simulink model "Ex-14050714-02_Hamming_Simulimk"  (R2025b)
settings: Solver=VariableStepDiscrete  StartTime=0.0  StopTime=1000  RelTol=1e-3
libraries: commblkcod2 x2, commrandsrc3 x1, commchan3 x1, commsink2 x1
settings Model: Creator=Pinnacle  LastModifiedBy=Pinnacle
settings SolverCC: AlgebraicLoopSolver=TrustRegion
settings DataIOCC: LimitDataPoints=on  SaveOutput=off  SaveTime=off
settings OptimizationCC: BooleanDataType=off  DefaultParameterBehavior=Inlined  LocalBlockOutputs=off  LifeSpan=inf
settings DebuggingCC: AlgebraicLoopMsg=error  SingleTaskRateTransMsg=error  UnconnectedInputMsg=warning  UnconnectedOutputMsg=warning  UnconnectedLineMsg=warning  AllowSymbolicDim=off  SFUnexpectedBacktrackingDiag=warning  SFNoUnconditionalDefaultTransitionDiag=warning  SFExecutionAtInitializationDiag=none  ArithmeticOperatorsInVariantConditions=warning
settings ModelReferenceCC: EnableRefExpFcnMdlSchedulingChecks=on
settings SFSimCC: SimUseLocalCustomCode=off  CustomCodeUndefinedFunction=UseInterfaceOnly
settings RTWCC: RTWUseLocalCustomCode=off  GPUComputeCapability=3.5
settings CodeAppCC: StateflowObjectComments=on
settings GRTTargetCC: TargetLangStandard=C89/C90 (ANSI)
settings ConfigComp: CovMetricSettings=dw  CovSaveCumulativeToWorkspaceVar=on  CovSaveSingleToWorkspaceVar=on  CovExternalEMLEnable=off  CovSFcnEnable=off

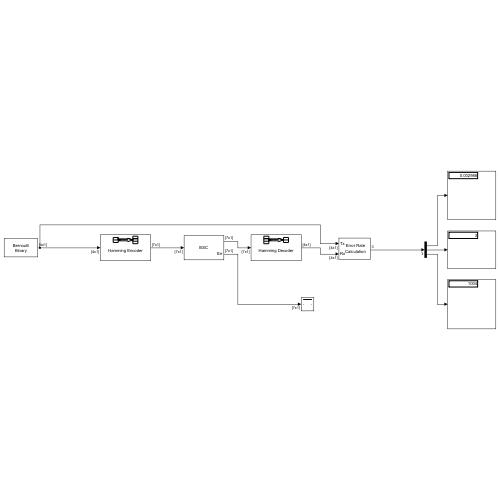
[thumbnail: Simulink's stored preview of the top-level diagram]
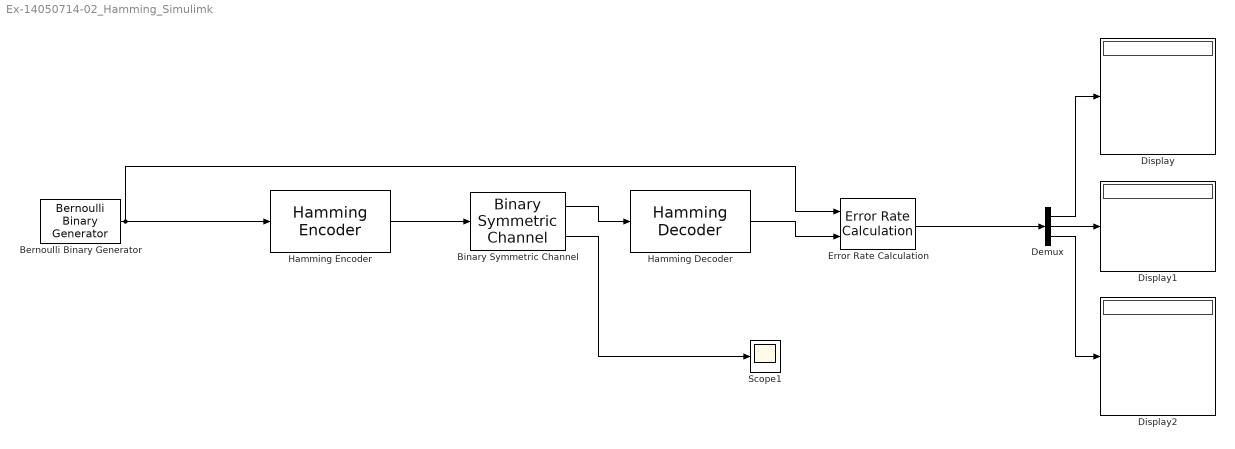
== system Ex-14050714-02_Hamming_Simulimk ==
  Bernoulli Binary Generator : commrandsrc3/Bernoulli Binary Generator  ProbabilityOfZero=0.5  SeedSource=Auto  Seed=0  SampleTime=1  SamplesPerFrame=4  OutputDataType=double  SimulateUsing=Interpreted execution
  Binary Symmetric Channel : commchan3/Binary Symmetric Channel  ErrorProbability=0.01  ErrorVectorOutputPort=on  OutputDataType=double  OutputDataTypeSL=double  Seed=71  SimulateUsing=Code generation
  Demux : Demux  Outputs=3
  Display : Display
  Display1 : Display
  Display2 : Display
  Error Rate Calculation : commsink2/Error Rate Calculation  N=0  st_delay=0  cp_mode=Entire frame  subframe=[]  PMode=Port  WsName=ErrorVec  RsMode2=off  stop=off  numErr=100  maxBits=1e6
  Hamming Decoder : commblkcod2/Hamming Decoder  n=7  k=4
  Hamming Encoder : commblkcod2/Hamming Encoder  n=7  k=4
  Scope1 : Scope
      settings: ActiveDisplayYMinimum=-0.12499999999999997  ActiveDisplayYMaximum=1.125
  wires:
  Bernoulli Binary Generator/1 -> Error Rate Calculation/1, Hamming Encoder/1
  Hamming Encoder/1 -> Binary Symmetric Channel/1
  Binary Symmetric Channel/2 -> Scope1/1
  Hamming Decoder/1 -> Error Rate Calculation/2
  Binary Symmetric Channel/1 -> Hamming Decoder/1
  Error Rate Calculation/1 -> Demux/1
  Demux/1 -> Display/1
  Demux/2 -> Display1/1
  Demux/3 -> Display2/1
